simulink model "AvonGasTurbineFAult"  (R2016b)
settings: Solver=ode45  StartTime=0.0  StopTime=3000  FixedStep=1  RelTol=1e-3  EnableMultiTasking=on
InitFcn:
  | warning off
undefined symbols (not defined in the file or in its folder): flagFalut, thresholdbound, xflt
libraries: neural x74, fuzblock x6, simulink x5
(part 1 of 4)
settings Model: Creator=Me  LastModifiedBy=Ali
settings DataIOCC: LimitDataPoints=on  SaveFormat=Array  SignalLoggingSaveFormat=ModelDataLogs
settings OptimizationCC: ExpressionDepthLimit=2147483647  LifeSpan=inf
settings DebuggingCC: UnderspecifiedInitializationDetection=Classic  MergeDetectMultiDrivingBlocksExec=none  SolverPrmCheckMsg=warning  FcnCallInpInsideContextMsg=warning  StateNameClashWarn=warning  SFUnexpectedBacktrackingDiag=warning  SFNoUnconditionalDefaultTransitionDiag=warning  SFExecutionAtInitializationDiag=none
settings HardwareCC: ProdBitPerPointer=32  ProdBitPerSizeT=32  ProdBitPerPtrDiffT=32  ProdLargestAtomicFloat=None  ProdIntDivRoundTo=Undefined  ProdEndianess=Unspecified  ProdWordSize=32  ProdHWDeviceType=32-bit Generic
settings ModelReferenceCC: PropagateSignalLabelsOutOfModel=off
settings GRTTargetCC: TargetLangStandard=C89/C90 (ANSI)  GeneratePreprocessorConditionals=Disable all  CombineOutputUpdateFcns=off  GRTInterface=on
settings ConfigComp: CovMetricSettings=dw  CovHtmlReporting=on  CovSaveCumulativeToWorkspaceVar=on  CovSaveSingleToWorkspaceVar=on  CovExternalEMLEnable=off  CovSFcnEnable=off
settings ConfigurationSet: Description=SimMechanics 2G

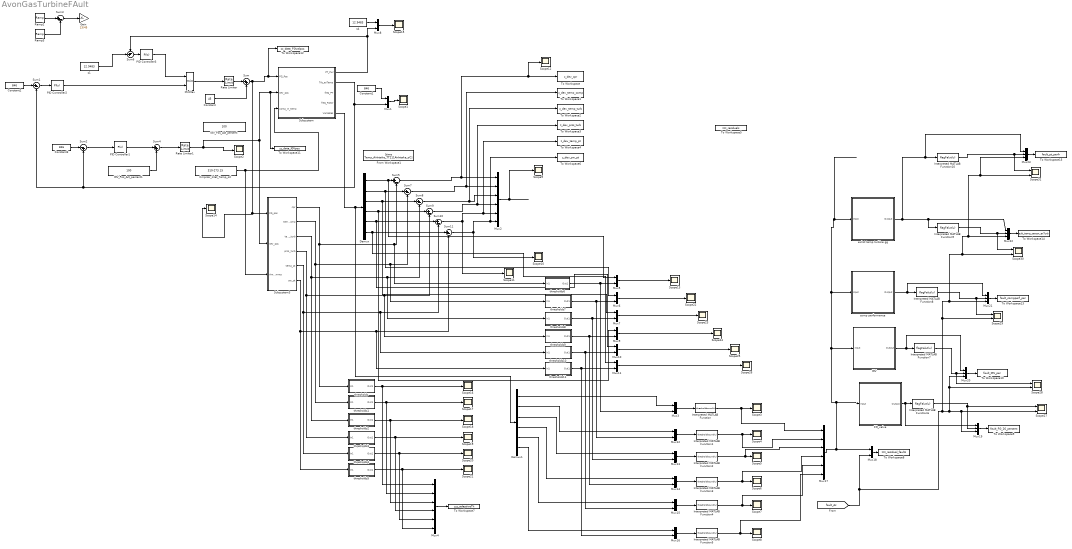
== system AvonGasTurbineFAult ==
  Cmprssr_Inlet_Temp_oC : Constant  Value=310-273.15
  Constant : Constant  Value=45
  Constant1 : Constant  Value=846
  Constant2 : Constant  Value=846
  Constant3 : Constant  Value=846
  Demux : Demux  Outputs=6
  Demux1 : Demux  Outputs=6
  FG_valve : Subsystem
      mask help: Pattern Recognition Neural Network
      mask Display: e = 0.06;c1 = [120 150 230]/255;c2 = ([120 150 230]+0)/383;c3 = ([120 150 230]+128)/383;patch([0 1 1 0],[0 0 1 1],c1);patch([0 1 1 1-e 1-e 0+e],[0 0 1 1-e 0+e 0+e],c2);patch([0 0 1 1-e 0+e 0+e],[0 1 1 1-e 1-e 0+e],c3);plot([0 1 1 0 0],[0 0 1 1 0]);fprintf('NNET');port_label('input',1,' Input');port_label('output',1,'Output ');
  From Workspace1 : FromWorkspace  VariableName="[time  Temp_AirIntake_TT211AirIntake_oC]"  SampleTime=0
  Gain : Gain  Gain=13/45
  IGV : Subsystem
      mask help: Pattern Recognition Neural Network
      mask Display: e = 0.06;c1 = [120 150 230]/255;c2 = ([120 150 230]+0)/383;c3 = ([120 150 230]+128)/383;patch([0 1 1 0],[0 0 1 1],c1);patch([0 1 1 1-e 1-e 0+e],[0 0 1 1-e 0+e 0+e],c2);patch([0 0 1 1-e 0+e 0+e],[0 1 1 1-e 1-e 0+e],c3);plot([0 1 1 0 0],[0 0 1 1 0]);fprintf('NNET');port_label('input',1,' Input');port_label('output',1,'Output ');
  IGV_Pos_Act_percent : Constant  Value=100
  IGV_Pos_Act_percent1 : Constant  Value=100
  Interpreted MATLAB Function{,1..5} (6 alike) : MATLABFcn  MATLABFcn=thresholdbound(u)  OutputDimensions=1
  Interpreted MATLAB Function{6..10} (5 alike) : MATLABFcn  MATLABFcn=flagFalut(u)  OutputDimensions=5
  MinMax : MinMax  Inputs=2
  Mux{1,3,5..16,18} (15 alike) : Mux  Inputs=2
  Mux17 : Mux  Inputs=6
  Mux{19..23} (5 alike) : Mux  Inputs=3
  Mux2 : Mux  Inputs=6
  Mux4 : Mux  Inputs=6
  PID Controller1 : simulink/Continuous/PID Controller  Controller=P  TimeDomain=Continuous-time  SampleTime=-1  IntegratorMethod=Forward Euler  FilterMethod=Forward Euler  Form=Ideal  UseFilter=on  ControllerParametersSource=internal  P=0.1  I=0.180070827922895  D=0  N=100  InitialConditionSource=internal  InitialConditionForIntegrator=0  InitialConditionForFilter=0  ExternalReset=none  LimitOutput=on  UpperSaturationLimit=15  LowerSaturationLimit=-100  LinearizeAsGain=on  AntiWindupMode=back-calculation  Kb=0.2  TrackingMode=off  Kt=1  PParamMin=[]  PParamMax=[]  IParamMin=[]  IParamMax=[]  DParamMin=[]  DParamMax=[]  NParamMin=[]  NParamMax=[]  KbParamMin=[]  KbParamMax=[]  KtParamMin=[]  KtParamMax=[]  POutMin=[]  POutMax=[]  IOutMin=[]  IOutMax=[]  DOutMin=[]  DOutMax=[]  NOutMin=[]  NOutMax=[]  KbOutMin=[]  KbOutMax=[]  KtOutMin=[]  KtOutMax=[]  IntegratorOutMin=[]  IntegratorOutMax=[]  FilterOutMin=[]  FilterOutMax=[]  SumOutMin=[]  SumOutMax=[]  SumI1OutMin=[]  SumI1OutMax=[]  SumI2OutMin=[]  SumI2OutMax=[]  SumI3OutMin=[]  SumI3OutMax=[]  SumDOutMin=[]  SumDOutMax=[]  SaturationOutMin=[]  SaturationOutMax=[]  IntegratorContinuousStateAttributes=''  IntegratorStateMustResolveToSignalObject=off  IntegratorRTWStateStorageClass=Auto  FilterContinuousStateAttributes=''  FilterStateMustResolveToSignalObject=off  FilterRTWStateStorageClass=Auto  DifferentiatorICPrevScaledInput=0  DifferentiatorOutMin=[]  DifferentiatorOutMax=[]
  PID Controller2 : simulink/Continuous/PID Controller  Controller=PI  TimeDomain=Continuous-time  SampleTime=-1  IntegratorMethod=Forward Euler  FilterMethod=Forward Euler  Form=Ideal  UseFilter=on  ControllerParametersSource=internal  P=0.0377674081389  I=0.180070827922895  D=0  N=100  InitialConditionSource=internal  InitialConditionForIntegrator=0  InitialConditionForFilter=0  ExternalReset=none  LimitOutput=on  UpperSaturationLimit=45  LowerSaturationLimit=-45  LinearizeAsGain=on  AntiWindupMode=back-calculation  Kb=0.2  TrackingMode=off  Kt=1  PParamMin=[]  PParamMax=[]  IParamMin=[]  IParamMax=[]  DParamMin=[]  DParamMax=[]  NParamMin=[]  NParamMax=[]  KbParamMin=[]  KbParamMax=[]  KtParamMin=[]  KtParamMax=[]  POutMin=[]  POutMax=[]  IOutMin=[]  IOutMax=[]  DOutMin=[]  DOutMax=[]  NOutMin=[]  NOutMax=[]  KbOutMin=[]  KbOutMax=[]  KtOutMin=[]  KtOutMax=[]  IntegratorOutMin=[]  IntegratorOutMax=[]  FilterOutMin=[]  FilterOutMax=[]  SumOutMin=[]  SumOutMax=[]  SumI1OutMin=[]  SumI1OutMax=[]  SumI2OutMin=[]  SumI2OutMax=[]  SumI3OutMin=[]  SumI3OutMax=[]  SumDOutMin=[]  SumDOutMax=[]  SaturationOutMin=[]  SaturationOutMax=[]  IntegratorContinuousStateAttributes=''  IntegratorStateMustResolveToSignalObject=off  IntegratorRTWStateStorageClass=Auto  FilterContinuousStateAttributes=''  FilterStateMustResolveToSignalObject=off  FilterRTWStateStorageClass=Auto  DifferentiatorICPrevScaledInput=0  DifferentiatorOutMin=[]  DifferentiatorOutMax=[]
  PID Controller3 : simulink/Continuous/PID Controller  Controller=PI  TimeDomain=Continuous-time  SampleTime=-1  IntegratorMethod=Forward Euler  FilterMethod=Forward Euler  Form=Ideal  UseFilter=on  ControllerParametersSource=internal  P=0.05  I=0.8  D=0  N=100  InitialConditionSource=internal  InitialConditionForIntegrator=0  InitialConditionForFilter=0  ExternalReset=none  LimitOutput=on  UpperSaturationLimit=60  LowerSaturationLimit=-30  LinearizeAsGain=on  AntiWindupMode=back-calculation  Kb=0.2  TrackingMode=off  Kt=1  PParamMin=[]  PParamMax=[]  IParamMin=[]  IParamMax=[]  DParamMin=[]  DParamMax=[]  NParamMin=[]  NParamMax=[]  KbParamMin=[]  KbParamMax=[]  KtParamMin=[]  KtParamMax=[]  POutMin=[]  POutMax=[]  IOutMin=[]  IOutMax=[]  DOutMin=[]  DOutMax=[]  NOutMin=[]  NOutMax=[]  KbOutMin=[]  KbOutMax=[]  KtOutMin=[]  KtOutMax=[]  IntegratorOutMin=[]  IntegratorOutMax=[]  FilterOutMin=[]  FilterOutMax=[]  SumOutMin=[]  SumOutMax=[]  SumI1OutMin=[]  SumI1OutMax=[]  SumI2OutMin=[]  SumI2OutMax=[]  SumI3OutMin=[]  SumI3OutMax=[]  SumDOutMin=[]  SumDOutMax=[]  SaturationOutMin=[]  SaturationOutMax=[]  IntegratorContinuousStateAttributes=''  IntegratorStateMustResolveToSignalObject=off  IntegratorRTWStateStorageClass=Auto  FilterContinuousStateAttributes=''  FilterStateMustResolveToSignalObject=off  FilterRTWStateStorageClass=Auto  DifferentiatorICPrevScaledInput=0  DifferentiatorOutMin=[]  DifferentiatorOutMax=[]
  Ramp2 : simulink/Sources/Ramp  slope=0.05  start=1000  X0=30
  Ramp3 : simulink/Sources/Ramp  slope=0.05  start=1300  X0=0
  Rate Limiter : RateLimiter  RisingSlewLimit=0.1  FallingSlewLimit=-0.1  SampleTimeMode=inherited  InitialCondition=45
  Rate Limiter1 : RateLimiter  RisingSlewLimit=0.1  FallingSlewLimit=-0.1  SampleTimeMode=inherited  InitialCondition=45
  Scope{1..26} (26 alike) : Scope
  Scope{27..31} (5 alike) : Scope  NumInputPorts=2
  Subsystem : Subsystem
  Subsystem3 : Subsystem
  Sum : Sum  Inputs=|++
  Sum{1,3,5,7..11} (8 alike) : Sum  Inputs=|+-
  Sum2 : Sum  Inputs=|-+
  Sum4 : Sum  Inputs=|++
  Sum6 : Sum  Inputs=-+|
  To Workspace : ToWorkspace  VariableName=z_dev_cpr  SampleTime=1
  To Workspace1 : ToWorkspace  VariableName=z_dev_temo_comp  SampleTime=1
  To Workspace10 : ToWorkspace  VariableName=fault_IGV_per  SampleTime=1
  To Workspace11 : ToWorkspace  VariableName=zz_data_IGVpos  SampleTime=1
  To Workspace12 : ToWorkspace  VariableName=zz_data_FGvalpos  SampleTime=1
  To Workspace13 : ToWorkspace  VariableName=fault_compperf_per  SampleTime=1
  To Workspace14 : ToWorkspace  VariableName=fault_temp_sensor_exTurb  SampleTime=1
  To Workspace15 : ToWorkspace  VariableName=fault_pt_perfr  SampleTime=1
  To Workspace2 : ToWorkspace  VariableName=z_dev_temp_turb  SampleTime=1
  To Workspace3 : ToWorkspace  VariableName=z_dev_prss_turb  SampleTime=1
  To Workspace4 : ToWorkspace  VariableName=z_dev_temp_pt  SampleTime=1
  To Workspace5 : ToWorkspace  VariableName=zzz_residuals  SampleTime=1
  To Workspace6 : ToWorkspace  VariableName=z_dev_pw_pt  SampleTime=1
  To Workspace7 : ToWorkspace  VariableName=zzz_adaptiveTh  SampleTime=1
  To Workspace8 : ToWorkspace  VariableName=zzz_residual_faults  SampleTime=1
  To Workspace9 : ToWorkspace  VariableName=fault_FG_26_percent  SampleTime=1
  comp performance : Subsystem
      mask help: Pattern Recognition Neural Network
      mask Display: e = 0.06;c1 = [120 150 230]/255;c2 = ([120 150 230]+0)/383;c3 = ([120 150 230]+128)/383;patch([0 1 1 0],[0 0 1 1],c1);patch([0 1 1 1-e 1-e 0+e],[0 0 1 1-e 0+e 0+e],c2);patch([0 0 1 1-e 0+e 0+e],[0 1 1 1-e 1-e 0+e],c3);plot([0 1 1 0 0],[0 0 1 1 0]);fprintf('NNET');port_label('input',1,' Input');port_label('output',1,'Output ');
  exhst temp turbine gg : Subsystem
      mask help: Pattern Recognition Neural Network
      mask Display: e = 0.06;c1 = [120 150 230]/255;c2 = ([120 150 230]+0)/383;c3 = ([120 150 230]+128)/383;patch([0 1 1 0],[0 0 1 1],c1);patch([0 1 1 1-e 1-e 0+e],[0 0 1 1-e 0+e 0+e],c2);patch([0 0 1 1-e 0+e 0+e],[0 1 1 1-e 1-e 0+e],c3);plot([0 1 1 0 0],[0 0 1 1 0]);fprintf('NNET');port_label('input',1,' Input');port_label('output',1,'Output ');
  s1 : Constant  Value=12.9483
  s4 : Constant  Value=12.9483
  thresholds : Subsystem
  thresholds1 : Subsystem
  thresholds10 : Subsystem
  thresholds11 : Subsystem
  thresholds2 : Subsystem
  thresholds3 : Subsystem
  thresholds4 : Subsystem
  thresholds5 : Subsystem
  thresholds6 : Subsystem
  thresholds7 : Subsystem
  thresholds8 : Subsystem
  thresholds9 : Subsystem
  wires:
  Ramp3/1 -> Sum3/2
  Ramp2/1 -> Sum3/1
  Subsystem/2(Trb_exTemp) -> Mux1/2, Sum2/2, Sum1/2
  Sum3/1 -> Gain/1
  Sum6/1 -> PID Controller3/1
  Sum1/1 -> PID Controller2/1
  Constant2/1 -> Sum1/1
  PID Controller2/1 -> MinMax/2
  MinMax/1 -> Rate Limiter/1
  PID Controller3/1 -> MinMax/1
  Mux8/1 -> Scope15/1
  s4/1 -> Mux8/1
  Subsystem/1(PT_Pwr) -> Sum6/1, Mux8/2
  Constant/1 -> Sum/2
  Sum/1 -> To Workspace12/1, Subsystem/1(FG_Pos), Scope14/1, Subsystem3/1(FG_pos)
  Rate Limiter/1 -> Sum/1
  Mux1/1 -> Scope1/1
  Constant1/1 -> Mux1/1
  Sum2/1 -> PID Controller1/1
  Constant3/1 -> Sum2/1
  PID Controller1/1 -> Sum4/1
  IGV_Pos_Act_percent1/1 -> Sum4/2
  Sum4/1 -> Rate Limiter1/1
  Rate Limiter1/1 -> Subsystem3/2(IGV_pos), To Workspace11/1, Subsystem/2(IGV_pos), Scope2/1
  Cmprssr_Inlet_Temp_oC/1 -> Subsystem3/3(Amb_Temmp), Subsystem/3(comp_in_temp)
  Subsystem3/2(temp_comp) -> thresholds7/1(In1), Sum7/2, thresholds1/1(In1)
  Subsystem3/5(temp_pt) -> thresholds10/1(In1), Sum10/2, thresholds4/1(In1)
  Subsystem3/6(pw_pt) -> thresholds11/1(In1), Sum11/2, thresholds5/1(In1)
  Subsystem/5(Variables) -> Demux1/1, Demux/1
  Demux/1 -> Mux5/1, Sum5/1
  Demux/4 -> Mux9/1, Sum9/1
  Demux/3 -> Mux7/1, Sum8/1
  Demux/2 -> Mux6/1, Sum7/1
  Demux/6 -> Mux11/1, Sum11/1
  Subsystem3/3(temp_turb) -> thresholds8/1(In1), Sum8/2, thresholds2/1(In1)
  Sum5/1 -> Mux2/1, Scope12/1, To Workspace/1
  Sum7/1 -> Mux2/2, To Workspace1/1
  Sum8/1 -> To Workspace2/1, Mux2/3
  Sum9/1 -> To Workspace3/1, Mux2/4
  Sum11/1 -> Scope10/1, To Workspace6/1, Mux2/6
  Mux2/1 -> Scope9/1
  Sum10/1 -> Scope11/1, To Workspace4/1, Mux2/5
  Subsystem3/1(cpr) -> Sum5/2, thresholds6/1(In1), thresholds/1(In1)
  s1/1 -> Sum6/2
  thresholds/1(Out1) -> Mux4/1, Scope16/1
  thresholds4/1(Out1) -> Mux4/5, Scope20/1
  thresholds3/1(Out1) -> Mux4/4, Scope19/1
  thresholds2/1(Out1) -> Mux4/3, Scope18/1
  thresholds1/1(Out1) -> Mux4/2, Scope17/1
  Mux4/1 -> To Workspace7/1
  Demux1/1 -> Mux3/1
  thresholds5/1(Out1) -> Mux4/6, Scope21/1
  Subsystem3/4(prss_turb) -> thresholds9/1(In1), Sum9/2, thresholds3/1(In1)
  thresholds6/1(Out1) -> Mux3/2, Mux5/2
  thresholds11/1(Out1) -> Mux16/2, Mux11/2
  thresholds10/1(Out1) -> Mux15/2, Mux10/2
  thresholds9/1(Out1) -> Mux14/2, Mux9/2
  thresholds8/1(Out1) -> Mux13/2, Mux7/2
  thresholds7/1(Out1) -> Mux12/2, Mux6/2
  Demux/5 -> Mux10/1, Sum10/1
  Mux5/1 -> Scope13/1
  Mux6/1 -> Scope22/1
  Mux7/1 -> Scope23/1
  Mux9/1 -> Scope24/1
  Mux10/1 -> Scope25/1
  Mux11/1 -> Scope26/1
  Demux1/2 -> Mux12/1
  Demux1/3 -> Mux13/1
  Demux1/4 -> Mux14/1
  Demux1/5 -> Mux15/1
  Demux1/6 -> Mux16/1
  Interpreted MATLAB Function1/1 -> Mux17/2, Scope4/1
  Interpreted MATLAB Function2/1 -> Mux17/3, Scope5/1
  Interpreted MATLAB Function3/1 -> Mux17/4, Scope6/1
  Interpreted MATLAB Function4/1 -> Mux17/5, Scope7/1
  Interpreted MATLAB Function5/1 -> Mux17/6, Scope8/1
  Interpreted MATLAB Function/1 -> Mux17/1, Scope3/1
  Mux3/1 -> Interpreted MATLAB Function/1
  Mux12/1 -> Interpreted MATLAB Function1/1
  Mux13/1 -> Interpreted MATLAB Function2/1
  Mux14/1 -> Interpreted MATLAB Function3/1
  Mux15/1 -> Interpreted MATLAB Function4/1
  Mux16/1 -> Interpreted MATLAB Function5/1
  Mux18/1 -> To Workspace8/1
  FG_valve/1(Output) -> Mux19/1, Interpreted MATLAB Function6/1
  Mux17/1 -> Mux18/1, FG_valve/1(Input), IGV/1(Input), exhst temp turbine gg/1(Input), comp performance/1(Input)
  Interpreted MATLAB Function6/1 -> Mux19/2, Scope27/1
  Mux19/1 -> To Workspace9/1
  IGV/1(Output) -> Mux20/1, Interpreted MATLAB Function7/1
  Mux20/1 -> To Workspace10/1
  Interpreted MATLAB Function7/1 -> Scope28/1, Mux20/2
  comp performance/1(Output) -> Mux21/1, Interpreted MATLAB Function8/1
  Mux21/1 -> To Workspace13/1
  Interpreted MATLAB Function8/1 -> Scope29/1, Mux21/2
  Mux22/1 -> To Workspace14/1
  Interpreted MATLAB Function9/1 -> Mux22/2, Scope30/1
  exhst temp turbine gg/1(Output) -> Interpreted MATLAB Function10/1, Mux23/1, Interpreted MATLAB Function9/1, Mux22/1
  Mux23/1 -> To Workspace15/1
  [fault_Ac] -> Scope29/2, Scope31/2, Mux23/3, Mux22/3, Scope30/2, Mux21/3, Scope28/2, Mux20/3, Mux19/3, Scope27/2, Mux18/2
  Interpreted MATLAB Function10/1 -> Scope31/1, Mux23/2

== system AvonGasTurbineFAult/FG_valve ==
  Input : Inport  PortDimensions=6
      mask Display: e = 0.06;c1 = [120 230 180]/255;c2 = ([120 230 180]+0)/(256+128);c3 = ([120 230 180]+128)/(256+128);patch([0 1 1 0],[0 0 1 1],c1);patch([0 1 1 1-e 1-e 0+e],[0 0 1 1-e 0+e 0+e],c2);patch([0 0 1 1-e 0+e 0+e],[0 1 1 1-e 1-e 0+e],c3);plot([0 1 1 0 0],[0 0 1 1 0]);
  Layer 1 : Subsystem
      mask Display: e = 0.06;c1 = [120 150 230]/255;c2 = ([120 150 230]+0)/383;c3 = ([120 150 230]+128)/383;patch([0 1 1 0],[0 0 1 1],c1);patch([0 1 1 1-e 1-e 0+e],[0 0 1 1-e 0+e 0+e],c2);patch([0 0 1 1-e 0+e 0+e],[0 1 1 1-e 1-e 0+e],c3);plot([0 1 1 0 0],[0 0 1 1 0]);
  Layer 2 : Subsystem
      mask Display: e = 0.06;c1 = [120 150 230]/255;c2 = ([120 150 230]+0)/383;c3 = ([120 150 230]+128)/383;patch([0 1 1 0],[0 0 1 1],c1);patch([0 1 1 1-e 1-e 0+e],[0 0 1 1-e 0+e 0+e],c2);patch([0 0 1 1-e 0+e 0+e],[0 1 1 1-e 1-e 0+e],c3);plot([0 1 1 0 0],[0 0 1 1 0]);
  Process Input 1 : Subsystem
      mask Display: e = 0.06;c1 = [120 150 230]/255;c2 = ([120 150 230]+0)/383;c3 = ([120 150 230]+128)/383;patch([0 1 1 0],[0 0 1 1],c1);patch([0 1 1 1-e 1-e 0+e],[0 0 1 1-e 0+e 0+e],c2);patch([0 0 1 1-e 0+e 0+e],[0 1 1 1-e 1-e 0+e],c3);plot([0 1 1 0 0],[0 0 1 1 0]);
  Process Output 1 : Subsystem
      mask Display: e = 0.06;c1 = [120 150 230]/255;c2 = ([120 150 230]+0)/383;c3 = ([120 150 230]+128)/383;patch([0 1 1 0],[0 0 1 1],c1);patch([0 1 1 1-e 1-e 0+e],[0 0 1 1-e 0+e 0+e],c2);patch([0 0 1 1-e 0+e 0+e],[0 1 1 1-e 1-e 0+e],c3);plot([0 1 1 0 0],[0 0 1 1 0]);
  Output : Outport  InitialOutput=[0;0;0;0;0]
      mask Display: e = 0.06;c1 = [120 230 180]/255;c2 = ([120 230 180]+0)/(256+128);c3 = ([120 230 180]+128)/(256+128);patch([0 1 1 0],[0 0 1 1],c1);patch([0 1 1 1-e 1-e 0+e],[0 0 1 1-e 0+e 0+e],c2);patch([0 0 1 1-e 0+e 0+e],[0 1 1 1-e 1-e 0+e],c3);plot([0 1 1 0 0],[0 0 1 1 0]);
  wires:
  Input/1 -> Process Input 1/1(x)
  Process Output 1/1(y) -> Output/1
  Process Input 1/1(p) -> Layer 1/1("p{1}")
  Layer 1/1("a{1}") -> [feedback1]
  [feedback1] -> Layer 2/1("a{1} ")
  Layer 2/1("a{2}") -> Process Output 1/1(a)

== system AvonGasTurbineFAult/IGV ==
  Input : Inport  PortDimensions=6
      mask Display: e = 0.06;c1 = [120 230 180]/255;c2 = ([120 230 180]+0)/(256+128);c3 = ([120 230 180]+128)/(256+128);patch([0 1 1 0],[0 0 1 1],c1);patch([0 1 1 1-e 1-e 0+e],[0 0 1 1-e 0+e 0+e],c2);patch([0 0 1 1-e 0+e 0+e],[0 1 1 1-e 1-e 0+e],c3);plot([0 1 1 0 0],[0 0 1 1 0]);
  Layer 1 : Subsystem
      mask Display: e = 0.06;c1 = [120 150 230]/255;c2 = ([120 150 230]+0)/383;c3 = ([120 150 230]+128)/383;patch([0 1 1 0],[0 0 1 1],c1);patch([0 1 1 1-e 1-e 0+e],[0 0 1 1-e 0+e 0+e],c2);patch([0 0 1 1-e 0+e 0+e],[0 1 1 1-e 1-e 0+e],c3);plot([0 1 1 0 0],[0 0 1 1 0]);
  Layer 2 : Subsystem
      mask Display: e = 0.06;c1 = [120 150 230]/255;c2 = ([120 150 230]+0)/383;c3 = ([120 150 230]+128)/383;patch([0 1 1 0],[0 0 1 1],c1);patch([0 1 1 1-e 1-e 0+e],[0 0 1 1-e 0+e 0+e],c2);patch([0 0 1 1-e 0+e 0+e],[0 1 1 1-e 1-e 0+e],c3);plot([0 1 1 0 0],[0 0 1 1 0]);
  Process Input 1 : Subsystem
      mask Display: e = 0.06;c1 = [120 150 230]/255;c2 = ([120 150 230]+0)/383;c3 = ([120 150 230]+128)/383;patch([0 1 1 0],[0 0 1 1],c1);patch([0 1 1 1-e 1-e 0+e],[0 0 1 1-e 0+e 0+e],c2);patch([0 0 1 1-e 0+e 0+e],[0 1 1 1-e 1-e 0+e],c3);plot([0 1 1 0 0],[0 0 1 1 0]);
  Process Output 1 : Subsystem
      mask Display: e = 0.06;c1 = [120 150 230]/255;c2 = ([120 150 230]+0)/383;c3 = ([120 150 230]+128)/383;patch([0 1 1 0],[0 0 1 1],c1);patch([0 1 1 1-e 1-e 0+e],[0 0 1 1-e 0+e 0+e],c2);patch([0 0 1 1-e 0+e 0+e],[0 1 1 1-e 1-e 0+e],c3);plot([0 1 1 0 0],[0 0 1 1 0]);
  Output : Outport  InitialOutput=[0;0;0;0;0]
      mask Display: e = 0.06;c1 = [120 230 180]/255;c2 = ([120 230 180]+0)/(256+128);c3 = ([120 230 180]+128)/(256+128);patch([0 1 1 0],[0 0 1 1],c1);patch([0 1 1 1-e 1-e 0+e],[0 0 1 1-e 0+e 0+e],c2);patch([0 0 1 1-e 0+e 0+e],[0 1 1 1-e 1-e 0+e],c3);plot([0 1 1 0 0],[0 0 1 1 0]);
  wires:
  Input/1 -> Process Input 1/1(x)
  Process Output 1/1(y) -> Output/1
  Process Input 1/1(p) -> Layer 1/1("p{1}")
  Layer 1/1("a{1}") -> [feedback1]
  [feedback1] -> Layer 2/1("a{1} ")
  Layer 2/1("a{2}") -> Process Output 1/1(a)

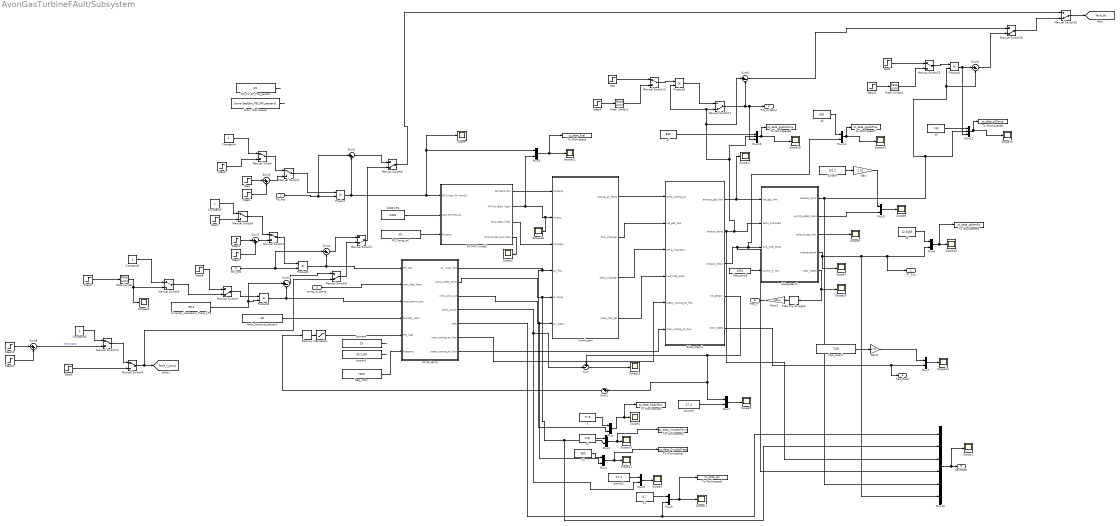
== system AvonGasTurbineFAult/Subsystem ==
  FG_Pos : Inport
  IGV_pos : Inport  Port=2
  comp_in_temp : Inport  Port=3
  2400 kPa : Constant  Value=2400
  Amb_Moisture_percent : Constant  Value=65
  Cmprssr_Upstream_Press_kPa : Constant  Value=99.2
  Combustor : Subsystem
  Constant{2..5} (4 alike) : Constant
  ExhaPr : Constant  Value=101.2
  FG MCV model : Subsystem
  FG_CV_SP_Pos_percen : Constant  Value=45
  FG_Temp_oC : Constant  Value=20
  From Workspace : FromWorkspace  VariableName=[time GasGen_PID_MV_percent]  SampleTime=0
  Gain : Gain  Gain=2.01
  Gain1 : Gain  Gain=30/pi
  Gain2 : Gain  Gain=pi/30
  Manual Switch{,1..2,4..5,9,12..13,15} (9 alike) : ManualSwitch
  Manual Switch{3,6..8,10..11,16} (7 alike) : ManualSwitch  CurrentSetting=0
  Memory : Memory  X0=28.945
  Memory Omega2 : Memory  X0=pi/30*4901
  Mux{,1..9,11} (11 alike) : Mux  Inputs=2
  Mux10 : Mux  Inputs=3
  Mux12 : Mux  Inputs=3
  Mux13 : Mux  Inputs=6
  Product{,1..4} (5 alike) : Product
  Rate Limiter : RateLimiter  RisingSlewLimit=0.005  FallingSlewLimit=-0.005  SampleTimeMode=inherited
  Rate Limiter1 : RateLimiter  RisingSlewLimit=0.005  FallingSlewLimit=-0.005  SampleTimeMode=inherited
  Rate Limiter2 : RateLimiter  RisingSlewLimit=0.005  FallingSlewLimit=-0.005  SampleTimeMode=inherited
  Saturation : Saturate  UpperLimit=40  LowerLimit=1
  Scope{,1..4,6..23} (23 alike) : Scope
  Step{,2..3,5,9,11} (6 alike) : Step  Time=1500  Before=1  After=1-xflt  SampleTime=0
  Step1 : Step  Time=1700  After=xflt  SampleTime=0
  Step10 : Step  Time=1200  Before=1  After=0.97  SampleTime=0
  Step12 : Step  Time=2000  After=-0.02  SampleTime=0
  Step4 : Step  Time=1700  After=xflt  SampleTime=0
  Step6 : Step  Time=1500  Before=1  After=0.976  SampleTime=0
  Step7 : Step  Time=1200  Before=1  After=1-0.09  SampleTime=0
  Step8 : Step  Time=1200  Before=1  After=1-0.07  SampleTime=0
  Subsystem1 : Subsystem
  Subsystem2 : Subsystem
  Sum : Sum  Inputs=+-|
  Sum1 : Sum  Inputs=-+|
  Sum{2,4..6,9} (5 alike) : Sum  Inputs=|+-
  Sum3 : Sum  Inputs=|++
  Sum7 : Sum  Inputs=|++
  Sum8 : Sum  Inputs=|++
  To Workspace : ToWorkspace  VariableName=zz_data_fuel  SampleTime=1
  To Workspace1 : ToWorkspace  VariableName=zz_data_cpr  SampleTime=1
  To Workspace2 : ToWorkspace  VariableName=zz_data_CmpdisPress  SampleTime=1
  To Workspace3 : ToWorkspace  VariableName=zz_data_CmpdisTemp  SampleTime=1
  To Workspace4 : ToWorkspace  VariableName=zz_data_trbAirflow  SampleTime=1
  To Workspace5 : ToWorkspace  VariableName=zz_data_ptGenPw  SampleTime=1
  To Workspace6 : ToWorkspace  VariableName=zz_data_ggdisTemp  SampleTime=1
  To Workspace7 : ToWorkspace  VariableName=zz_data_ggdisPres  SampleTime=1
  To Workspace8 : ToWorkspace  VariableName=zz_data_ptTemp  SampleTime=1
  comp_temp : Subsystem
  freq_pwtrb : Constant  Value=4901
  freq_rotor : Constant  Value=7250
  freq_rotor1 : Constant  Value=7250
  power2 : Constant  Value=27.4
  power4 : Constant  Value=25
  power5 : Constant  Value=26.2350
  power6 : Constant  Value=27.4
  s : Constant  Value=77.8
  s1 : Constant  Value=9.7
  s2 : Constant  Value=378
  s3 : Constant  Value=960
  s4 : Constant  Value=12.9483
  s7 : Constant  Value=846
  s8 : Constant  Value=335
  s9 : Constant  Value=745
  test : Step  Time=1200  Before=1  After=0.95  SampleTime=0
  test1 : Step  Time=1200  Before=1  After=0.95  SampleTime=0
  PT_Pwr : Outport
  Trb_exTemp : Outport  Port=2
  freq_PT : Outport  Port=3
  freq_Rotor : Outport  Port=4
  Variables : Outport  Port=5
  tag scope: fault_Ac=global, fault_f_comp=global
  wires:
  FG_CV_SP_Pos_percen/1 -> ?
  From Workspace/1 -> ?
  Gain1/1 -> freq_PT/1
  power5/1 -> ?
  power4/1 -> ?
  Amb_Moisture_percent/1 -> comp_temp/4(humidity_ratio)
  freq_rotor/1 -> comp_temp/6(Frequency)
  IGV_pos/1 -> Product1/2, Sum4/1
  Subsystem1/3(exhaust_gas_flow) -> Scope6/1
  Memory/1 -> Saturation/1
  FG_Temp_oC/1 -> FG MCV model/3(FG temp.)
  comp_temp/3(comp_prss_out) -> Mux4/2, Combustor/6(air_press)
  FG MCV model/2(FG Flow @bur (kg/s)) -> Mux9/2, Scope16/1, Combustor/2(FG flow)
  Combustor/2(flow_chamber) -> Subsystem2/2(hot_gas_flow)
  comp_temp/4(comp_power) -> Mux5/2, Sum/2
  Mux1/1 -> Scope9/1
  Mux6/1 -> To Workspace1/1, Scope11/1
  comp_temp/5(CPR) -> Mux13/1, Mux6/2
  Mux4/1 -> To Workspace2/1, Scope12/1
  FG MCV model/1(FG Temp (oC)) -> Combustor/1(FG temp)
  Mux2/1 -> To Workspace3/1, Scope10/1
  2400 kPa/1 -> FG MCV model/2(main FG line prss)
  ExhaPr/1 -> Gain/1
  Combustor/1(cooling_air_temp) -> Subsystem2/1(temp_cooling_air)
  FG MCV model/3(FG pr @bur (kPa)) -> Combustor/3(FG press)
  Subsystem2/3(exhaust_press) -> Mux13/4, Subsystem1/3(turb_inlet_press), Mux11/2
  Combustor/3(temp_chamber) -> Subsystem2/3(temp_chambers)
  FG MCV model/4(FG skid inlet prss (kPa)) -> Scope2/1
  Subsystem2/1(exhaust_gas_flow) -> Subsystem1/1(hot_gas_flow), Scope17/1
  Subsystem1/2(pwrtrb_outlet_press) -> Mux3/2
  power6/1 -> Mux1/2
  Gain/1 -> Mux3/1
  Mux3/1 -> Scope8/1
  comp_temp/1(air_mass_flow) -> Combustor/4(air_flow), Mux/2
  comp_temp/2(comp_outlet_temp) -> Mux13/2, Mux2/2, Combustor/5(air temp)
  Combustor/4(press_hot_gas) -> Subsystem2/4(turb_inlet_press)
  Mux8/1 -> To Workspace5/1, Scope15/1
  Mux7/1 -> Scope14/1
  Product/1 -> Mux9/1, Scope/1, FG MCV model/1(FG CV pos (%) chmb1), Sum2/2
  Subsystem1/4(turbine_power) -> Mux13/6, PT_Pwr/1, Mux8/2, Scope7/1
  comp_temp/7(stator_cooling_air_flow) -> Subsystem2/6(rotor_cooling_air_flow)
  Mux11/1 -> To Workspace7/1, Scope22/1
  s2/1 -> Mux2/1
  Sum1/1 -> Memory/1
  Mux9/1 -> To Workspace/1, Scope21/1
  Mux/1 -> To Workspace4/1, Scope4/1
  s/1 -> Mux/1
  s7/1 -> Mux10/1
  s1/1 -> Mux6/1
  Mux10/1 -> Scope18/1, To Workspace6/1
  Mux5/1 -> Scope3/1
  Sum/1 -> Scope13/1
  Subsystem2/5(rotor_speed) -> freq_Rotor/1, Mux7/2
  comp_temp/6(rotor_cooling_air_flow) -> Subsystem2/5(stator_cooling_air_flow)
  s3/1 -> Mux4/1
  freq_pwtrb/1 -> Subsystem1/4(pwrtrb_fr_rpm)
  power2/1 -> Mux5/1
  Subsystem1/5(rotor_speed) -> Scope20/1, Memory Omega2/1
  Gain2/1 -> Mux7/1
  Saturation/1 -> comp_temp/5(MW_load)
  Memory Omega2/1 -> Gain1/1
  freq_rotor1/1 -> Gain2/1
  Subsystem2/4(trb_genpwr) -> Sum/1, Sum1/2, Mux1/1
  s4/1 -> Mux8/1
  s9/1 -> Mux12/1
  s8/1 -> Mux11/1
  Mux12/1 -> To Workspace8/1, Scope19/1
  comp_in_temp/1 -> comp_temp/2(cmp_Inlet_Temp)
  FG_Pos/1 -> Sum2/1, Product/2
  Mux13/1 -> Scope1/1, Variables/1
  Sum2/1 -> Manual Switch6/1
  Step/1 -> Sum3/1
  Step1/1 -> Sum3/2
  Product1/1 -> Sum4/2, comp_temp/1(IGV_pos)
  Manual Switch5/1 -> Manual Switch2/1
  Cmprssr_Upstream_Press_kPa/1 -> Sum5/1, Product2/2
  Product2/1 -> Sum5/2, comp_temp/3(cmp_upstrm_prss)
  Step2/1 -> Rate Limiter/1
  Rate Limiter/1 -> Manual Switch9/2, Scope23/1
  Step3/1 -> Sum7/1
  Step4/1 -> Sum7/2
  Manual Switch3/1 -> Product2/1
  Constant3/1 -> Manual Switch12/1
  Step6/1 -> Manual Switch/2
  Sum3/1 -> Manual Switch1/2
  Manual Switch/1 -> Manual Switch1/1
  Constant4/1 -> Manual Switch/1
  Manual Switch1/1 -> Product/1
  Manual Switch2/1 -> Product1/1
  Sum7/1 -> Manual Switch2/2
  Step8/1 -> Manual Switch3/1
  Manual Switch4/1 -> Manual Switch8/2, [fault_f_comp]
  Step5/1 -> Manual Switch4/2
  Step7/1 -> Manual Switch5/2
  Constant5/1 -> Manual Switch5/1
  Manual Switch7/1 -> Manual Switch6/2
  Manual Switch6/1 -> Manual Switch10/1
  Sum4/1 -> Manual Switch7/1
  Sum5/1 -> Manual Switch8/1
  Manual Switch8/1 -> Manual Switch7/2
  Manual Switch9/1 -> Manual Switch3/2
  Constant2/1 -> Manual Switch9/1
  Manual Switch10/1 -> [fault_Ac]
  Sum6/1 -> Manual Switch16/1
  Rate Limiter1/1 -> Manual Switch13/2
  Product3/1 -> Manual Switch11/1
  Subsystem2/2(exhaust_temp) -> Mux13/3, Sum6/1, Manual Switch11/2, Product3/2, Mux10/2, Subsystem1/2(temp_chambers)
  Manual Switch11/1 -> Mux10/3, Trb_exTemp/1, Sum6/2
  Manual Switch12/1 -> Manual Switch4/1
  Manual Switch13/1 -> Product3/1
  test/1 -> Manual Switch13/1
  Step10/1 -> Sum8/1
  Step12/1 -> Sum8/2
  Sum8/1 -> Manual Switch12/2  "test signal"
  Step9/1 -> Rate Limiter1/1
  Manual Switch16/1 -> Manual Switch10/2
  Rate Limiter2/1 -> Manual Switch15/2
  Product4/1 -> Mux12/3, Sum9/1
  Subsystem1/1(exhaust_temp) -> Mux12/2, Sum9/2, Product4/2, Mux13/5
  Manual Switch15/1 -> Product4/1
  test1/1 -> Manual Switch15/1
  Step11/1 -> Rate Limiter2/1
  Sum9/1 -> Manual Switch16/2

== system AvonGasTurbineFAult/Subsystem3 ==
  FG_pos : Inport
  IGV_pos : Inport  Port=2
  Amb_Temmp : Inport  Port=3
  CPR : fuzblock/Fuzzy Logic  Controller  fis=readfis('fis_CPR')
  Gain1 : Gain  Gain=11.0390
  Gain10 : Gain  Gain=1/115
  Gain11 : Gain  Gain=1/40
  Gain12 : Gain  Gain=888.3645
  Gain13 : Gain  Gain=381.1970
  Gain14 : Gain  Gain=779.6646
  Gain15 : Gain  Gain=17.9878
  Gain2 : Gain  Gain=382.2652
  Gain3 : Gain  Gain=1/6.6359
  Gain9 : Gain  Gain=1/50
  Laguerre3 : Subsystem  mask{a1=0.96, fltrordr=5, smp=1}
      mask prompts: a1 "Laguerre pole"; fltrordr "filter order (n=L+1)"; smp "sample time"
      mask Display: disp('Laguerre Filter')
  Laguerre4 : Subsystem  mask{a1=0.96, fltrordr=5, smp=1}
      mask prompts: a1 "Laguerre pole"; fltrordr "filter order (n=L+1)"; smp "sample time"
      mask Display: disp('Laguerre Filter')
  Laguerre5 : Subsystem  mask{a1=0.96, fltrordr=5, smp=1}
      mask prompts: a1 "Laguerre pole"; fltrordr "filter order (n=L+1)"; smp "sample time"
      mask Display: disp('Laguerre Filter')
  Mux22 : Mux  Inputs=3
  power_pt : fuzblock/Fuzzy Logic  Controller  fis=readfis('fis_power_pt')
  prss_turb1 : fuzblock/Fuzzy Logic  Controller  fis=readfis('fis_prss_turb')
  temp_comp1 : fuzblock/Fuzzy Logic  Controller  fis=readfis('fis_temp_comp')
  temp_pt1 : fuzblock/Fuzzy Logic  Controller  fis=readfis('fis_temp_pt')
  temp_turb1 : fuzblock/Fuzzy Logic  Controller  fis=readfis('fis_temp_turb')
  cpr : Outport
  temp_comp : Outport  Port=2
  temp_turb : Outport  Port=3
  prss_turb : Outport  Port=4
  temp_pt : Outport  Port=5
  pw_pt : Outport  Port=6
  wires:
  IGV_pos/1 -> Gain10/1
  Gain10/1 -> Laguerre4/1(u)
  Laguerre5/1(v) -> Mux22/3
  Gain9/1 -> Laguerre3/1(u)
  Laguerre3/1(v) -> Mux22/1
  Gain11/1 -> Laguerre5/1(u)
  Mux22/1 -> Gain3/1
  Laguerre4/1(v) -> Mux22/2
  FG_pos/1 -> Gain9/1
  Amb_Temmp/1 -> Gain11/1
  Gain1/1 -> cpr/1
  Gain2/1 -> temp_comp/1
  Gain12/1 -> temp_turb/1
  Gain13/1 -> prss_turb/1
  Gain14/1 -> temp_pt/1
  Gain15/1 -> pw_pt/1
  temp_comp1/1 -> Gain2/1
  temp_turb1/1 -> Gain12/1
  prss_turb1/1 -> Gain13/1
  temp_pt1/1 -> Gain14/1
  power_pt/1 -> Gain15/1
  CPR/1 -> Gain1/1
  Gain3/1 -> temp_turb1/1, prss_turb1/1, temp_pt1/1, power_pt/1, temp_comp1/1, CPR/1

== system AvonGasTurbineFAult/comp performance ==
  Input : Inport  PortDimensions=6
      mask Display: e = 0.06;c1 = [120 230 180]/255;c2 = ([120 230 180]+0)/(256+128);c3 = ([120 230 180]+128)/(256+128);patch([0 1 1 0],[0 0 1 1],c1);patch([0 1 1 1-e 1-e 0+e],[0 0 1 1-e 0+e 0+e],c2);patch([0 0 1 1-e 0+e 0+e],[0 1 1 1-e 1-e 0+e],c3);plot([0 1 1 0 0],[0 0 1 1 0]);
  Layer 1 : Subsystem
      mask Display: e = 0.06;c1 = [120 150 230]/255;c2 = ([120 150 230]+0)/383;c3 = ([120 150 230]+128)/383;patch([0 1 1 0],[0 0 1 1],c1);patch([0 1 1 1-e 1-e 0+e],[0 0 1 1-e 0+e 0+e],c2);patch([0 0 1 1-e 0+e 0+e],[0 1 1 1-e 1-e 0+e],c3);plot([0 1 1 0 0],[0 0 1 1 0]);
  Layer 2 : Subsystem
      mask Display: e = 0.06;c1 = [120 150 230]/255;c2 = ([120 150 230]+0)/383;c3 = ([120 150 230]+128)/383;patch([0 1 1 0],[0 0 1 1],c1);patch([0 1 1 1-e 1-e 0+e],[0 0 1 1-e 0+e 0+e],c2);patch([0 0 1 1-e 0+e 0+e],[0 1 1 1-e 1-e 0+e],c3);plot([0 1 1 0 0],[0 0 1 1 0]);
  Process Input 1 : Subsystem
      mask Display: e = 0.06;c1 = [120 150 230]/255;c2 = ([120 150 230]+0)/383;c3 = ([120 150 230]+128)/383;patch([0 1 1 0],[0 0 1 1],c1);patch([0 1 1 1-e 1-e 0+e],[0 0 1 1-e 0+e 0+e],c2);patch([0 0 1 1-e 0+e 0+e],[0 1 1 1-e 1-e 0+e],c3);plot([0 1 1 0 0],[0 0 1 1 0]);
  Process Output 1 : Subsystem
      mask Display: e = 0.06;c1 = [120 150 230]/255;c2 = ([120 150 230]+0)/383;c3 = ([120 150 230]+128)/383;patch([0 1 1 0],[0 0 1 1],c1);patch([0 1 1 1-e 1-e 0+e],[0 0 1 1-e 0+e 0+e],c2);patch([0 0 1 1-e 0+e 0+e],[0 1 1 1-e 1-e 0+e],c3);plot([0 1 1 0 0],[0 0 1 1 0]);
  Output : Outport  InitialOutput=[0;0;0;0;0]
      mask Display: e = 0.06;c1 = [120 230 180]/255;c2 = ([120 230 180]+0)/(256+128);c3 = ([120 230 180]+128)/(256+128);patch([0 1 1 0],[0 0 1 1],c1);patch([0 1 1 1-e 1-e 0+e],[0 0 1 1-e 0+e 0+e],c2);patch([0 0 1 1-e 0+e 0+e],[0 1 1 1-e 1-e 0+e],c3);plot([0 1 1 0 0],[0 0 1 1 0]);
  wires:
  Input/1 -> Process Input 1/1(x)
  Process Output 1/1(y) -> Output/1
  Process Input 1/1(p) -> Layer 1/1("p{1}")
  Layer 1/1("a{1}") -> [feedback1]
  [feedback1] -> Layer 2/1("a{1} ")
  Layer 2/1("a{2}") -> Process Output 1/1(a)

== system AvonGasTurbineFAult/exhst temp turbine gg ==
  Input : Inport  PortDimensions=6
      mask Display: e = 0.06;c1 = [120 230 180]/255;c2 = ([120 230 180]+0)/(256+128);c3 = ([120 230 180]+128)/(256+128);patch([0 1 1 0],[0 0 1 1],c1);patch([0 1 1 1-e 1-e 0+e],[0 0 1 1-e 0+e 0+e],c2);patch([0 0 1 1-e 0+e 0+e],[0 1 1 1-e 1-e 0+e],c3);plot([0 1 1 0 0],[0 0 1 1 0]);
  Layer 1 : Subsystem
      mask Display: e = 0.06;c1 = [120 150 230]/255;c2 = ([120 150 230]+0)/383;c3 = ([120 150 230]+128)/383;patch([0 1 1 0],[0 0 1 1],c1);patch([0 1 1 1-e 1-e 0+e],[0 0 1 1-e 0+e 0+e],c2);patch([0 0 1 1-e 0+e 0+e],[0 1 1 1-e 1-e 0+e],c3);plot([0 1 1 0 0],[0 0 1 1 0]);
  Layer 2 : Subsystem
      mask Display: e = 0.06;c1 = [120 150 230]/255;c2 = ([120 150 230]+0)/383;c3 = ([120 150 230]+128)/383;patch([0 1 1 0],[0 0 1 1],c1);patch([0 1 1 1-e 1-e 0+e],[0 0 1 1-e 0+e 0+e],c2);patch([0 0 1 1-e 0+e 0+e],[0 1 1 1-e 1-e 0+e],c3);plot([0 1 1 0 0],[0 0 1 1 0]);
  Process Input 1 : Subsystem
      mask Display: e = 0.06;c1 = [120 150 230]/255;c2 = ([120 150 230]+0)/383;c3 = ([120 150 230]+128)/383;patch([0 1 1 0],[0 0 1 1],c1);patch([0 1 1 1-e 1-e 0+e],[0 0 1 1-e 0+e 0+e],c2);patch([0 0 1 1-e 0+e 0+e],[0 1 1 1-e 1-e 0+e],c3);plot([0 1 1 0 0],[0 0 1 1 0]);
  Process Output 1 : Subsystem
      mask Display: e = 0.06;c1 = [120 150 230]/255;c2 = ([120 150 230]+0)/383;c3 = ([120 150 230]+128)/383;patch([0 1 1 0],[0 0 1 1],c1);patch([0 1 1 1-e 1-e 0+e],[0 0 1 1-e 0+e 0+e],c2);patch([0 0 1 1-e 0+e 0+e],[0 1 1 1-e 1-e 0+e],c3);plot([0 1 1 0 0],[0 0 1 1 0]);
  Output : Outport  InitialOutput=[0;0;0;0;0]
      mask Display: e = 0.06;c1 = [120 230 180]/255;c2 = ([120 230 180]+0)/(256+128);c3 = ([120 230 180]+128)/(256+128);patch([0 1 1 0],[0 0 1 1],c1);patch([0 1 1 1-e 1-e 0+e],[0 0 1 1-e 0+e 0+e],c2);patch([0 0 1 1-e 0+e 0+e],[0 1 1 1-e 1-e 0+e],c3);plot([0 1 1 0 0],[0 0 1 1 0]);
  wires:
  Input/1 -> Process Input 1/1(x)
  Process Output 1/1(y) -> Output/1
  Process Input 1/1(p) -> Layer 1/1("p{1}")
  Layer 1/1("a{1}") -> [feedback1]
  [feedback1] -> Layer 2/1("a{1} ")
  Layer 2/1("a{2}") -> Process Output 1/1(a)

== system AvonGasTurbineFAult/thresholds ==
  In1 : Inport
  Constant5 : Constant  Value=0.0178
  Mux5 : Mux  Inputs=3
  Sum12 : Sum  Inputs=|++
  Sum13 : Sum  Inputs=|++
  Sum14 : Sum  Inputs=-+|
  var : Gain  Gain=0.0665
  var1 : Gain  Gain=0.2
  Out1 : Outport
  wires:
  var1/1 -> var/1
  Sum14/1 -> Mux5/3
  Sum13/1 -> Sum12/1, var1/1, Sum14/2
  var/1 -> Sum14/1, Sum12/2
  Mux5/1 -> Out1/1
  Sum12/1 -> Mux5/2
  Constant5/1 -> Sum13/2
  In1/1 -> Mux5/1, Sum13/1

== system AvonGasTurbineFAult/thresholds1 ==
  In1 : Inport
  Constant5 : Constant  Value=-2.9
  Mux5 : Mux  Inputs=3
  Sum12 : Sum  Inputs=|++
  Sum13 : Sum  Inputs=|++
  Sum14 : Sum  Inputs=-+|
  var : Gain  Gain=0.0069
  var1 : Gain  Gain=2.5
  Out1 : Outport
  wires:
  In1/1 -> Sum13/1, Mux5/1
  Constant5/1 -> Sum13/2
  Sum12/1 -> Mux5/2
  Mux5/1 -> Out1/1
  var/1 -> Sum12/2, Sum14/1
  Sum13/1 -> Sum14/2, var1/1, Sum12/1
  Sum14/1 -> Mux5/3
  var1/1 -> var/1

== system AvonGasTurbineFAult/thresholds10 ==
  In1 : Inport
  Constant5 : Constant  Value=-2.0766
  Mux5 : Mux  Inputs=2
  Sum12 : Sum  Inputs=|++
  Sum13 : Sum  Inputs=|++
  Sum14 : Sum  Inputs=-+|
  var : Gain  Gain=0.03
  var1 : Gain  Gain=0.19
  Out1 : Outport
  wires:
  var1/1 -> var/1
  Sum14/1 -> Mux5/2
  Sum13/1 -> Sum12/1, var1/1, Sum14/2
  var/1 -> Sum14/1, Sum12/2
  Mux5/1 -> Out1/1
  Sum12/1 -> Mux5/1
  Constant5/1 -> Sum13/2
  In1/1 -> Sum13/1

== system AvonGasTurbineFAult/thresholds11 ==
  In1 : Inport
  Constant5 : Constant  Value=0
  Mux5 : Mux  Inputs=2
  Sum12 : Sum  Inputs=|++
  Sum13 : Sum  Inputs=|++
  Sum14 : Sum  Inputs=-+|
  var : Gain  Gain=0.25
  var1 : Gain  Gain=0.22
  Out1 : Outport
  wires:
  In1/1 -> Sum13/1
  Constant5/1 -> Sum13/2
  Sum12/1 -> Mux5/1
  Mux5/1 -> Out1/1
  var/1 -> Sum12/2, Sum14/1
  Sum13/1 -> Sum14/2, var1/1, Sum12/1
  Sum14/1 -> Mux5/2
  var1/1 -> var/1

== system AvonGasTurbineFAult/thresholds2 ==
  In1 : Inport
  Constant5 : Constant  Value=0.05
  Mux5 : Mux  Inputs=3
  Sum12 : Sum  Inputs=|++
  Sum13 : Sum  Inputs=|++
  Sum14 : Sum  Inputs=-+|
  var : Gain  Gain=0.05
  var1 : Gain  Gain=0.19
  Out1 : Outport
  wires:
  var1/1 -> var/1
  Sum14/1 -> Mux5/3
  Sum13/1 -> Sum12/1, var1/1, Sum14/2
  var/1 -> Sum14/1, Sum12/2
  Mux5/1 -> Out1/1
  Sum12/1 -> Mux5/2
  Constant5/1 -> Sum13/2
  In1/1 -> Mux5/1, Sum13/1

== system AvonGasTurbineFAult/thresholds3 ==
  In1 : Inport
  Constant5 : Constant  Value=-0.3406
  Mux5 : Mux  Inputs=3
  Sum12 : Sum  Inputs=|++
  Sum13 : Sum  Inputs=|++
  Sum14 : Sum  Inputs=-+|
  var : Gain  Gain=0.01
  var1 : Gain  Gain=0.19
  Out1 : Outport
  wires:
  In1/1 -> Sum13/1, Mux5/1
  Constant5/1 -> Sum13/2
  Sum12/1 -> Mux5/2
  Mux5/1 -> Out1/1
  var/1 -> Sum12/2, Sum14/1
  Sum13/1 -> Sum14/2, var1/1, Sum12/1
  Sum14/1 -> Mux5/3
  var1/1 -> var/1

== system AvonGasTurbineFAult/thresholds4 ==
  In1 : Inport
  Constant5 : Constant  Value=-2.0766
  Mux5 : Mux  Inputs=3
  Sum12 : Sum  Inputs=|++
  Sum13 : Sum  Inputs=|++
  Sum14 : Sum  Inputs=-+|
  var : Gain  Gain=0.03
  var1 : Gain  Gain=0.19
  Out1 : Outport
  wires:
  var1/1 -> var/1
  Sum14/1 -> Mux5/3
  Sum13/1 -> Sum12/1, var1/1, Sum14/2
  var/1 -> Sum14/1, Sum12/2
  Mux5/1 -> Out1/1
  Sum12/1 -> Mux5/2
  Constant5/1 -> Sum13/2
  In1/1 -> Mux5/1, Sum13/1

== system AvonGasTurbineFAult/thresholds5 ==
  In1 : Inport
  Constant5 : Constant  Value=0
  Mux5 : Mux  Inputs=3
  Sum12 : Sum  Inputs=|++
  Sum13 : Sum  Inputs=|++
  Sum14 : Sum  Inputs=-+|
  var : Gain  Gain=0.25
  var1 : Gain  Gain=0.22
  Out1 : Outport
  wires:
  In1/1 -> Sum13/1, Mux5/1
  Constant5/1 -> Sum13/2
  Sum12/1 -> Mux5/2
  Mux5/1 -> Out1/1
  var/1 -> Sum12/2, Sum14/1
  Sum13/1 -> Sum14/2, var1/1, Sum12/1
  Sum14/1 -> Mux5/3
  var1/1 -> var/1

== system AvonGasTurbineFAult/thresholds6 ==
  In1 : Inport
  Constant5 : Constant  Value=0.0178
  Mux5 : Mux  Inputs=2
  Sum12 : Sum  Inputs=|++
  Sum13 : Sum  Inputs=|++
  Sum14 : Sum  Inputs=-+|
  var : Gain  Gain=0.0665
  var1 : Gain  Gain=0.2
  Out1 : Outport
  wires:
  var1/1 -> var/1
  Sum14/1 -> Mux5/2
  Sum13/1 -> Sum12/1, var1/1, Sum14/2
  var/1 -> Sum14/1, Sum12/2
  Mux5/1 -> Out1/1
  Sum12/1 -> Mux5/1
  Constant5/1 -> Sum13/2
  In1/1 -> Sum13/1

== system AvonGasTurbineFAult/thresholds7 ==
  In1 : Inport
  Constant5 : Constant  Value=-2.9
  Mux5 : Mux  Inputs=2
  Sum12 : Sum  Inputs=|++
  Sum13 : Sum  Inputs=|++
  Sum14 : Sum  Inputs=-+|
  var : Gain  Gain=0.0069
  var1 : Gain  Gain=2.5
  Out1 : Outport
  wires:
  In1/1 -> Sum13/1
  Constant5/1 -> Sum13/2
  Sum12/1 -> Mux5/1
  Mux5/1 -> Out1/1
  var/1 -> Sum12/2, Sum14/1
  Sum13/1 -> Sum14/2, var1/1, Sum12/1
  Sum14/1 -> Mux5/2
  var1/1 -> var/1

== system AvonGasTurbineFAult/thresholds8 ==
  In1 : Inport
  Constant5 : Constant  Value=0.05
  Mux5 : Mux  Inputs=2
  Sum12 : Sum  Inputs=|++
  Sum13 : Sum  Inputs=|++
  Sum14 : Sum  Inputs=-+|
  var : Gain  Gain=0.05
  var1 : Gain  Gain=0.19
  Out1 : Outport
  wires:
  var1/1 -> var/1
  Sum14/1 -> Mux5/2
  Sum13/1 -> Sum12/1, var1/1, Sum14/2
  var/1 -> Sum14/1, Sum12/2
  Mux5/1 -> Out1/1
  Sum12/1 -> Mux5/1
  Constant5/1 -> Sum13/2
  In1/1 -> Sum13/1

== system AvonGasTurbineFAult/thresholds9 ==
  In1 : Inport
  Constant5 : Constant  Value=-0.3406
  Mux5 : Mux  Inputs=2
  Sum12 : Sum  Inputs=|++
  Sum13 : Sum  Inputs=|++
  Sum14 : Sum  Inputs=-+|
  var : Gain  Gain=0.01
  var1 : Gain  Gain=0.19
  Out1 : Outport
  wires:
  In1/1 -> Sum13/1
  Constant5/1 -> Sum13/2
  Sum12/1 -> Mux5/1
  Mux5/1 -> Out1/1
  var/1 -> Sum12/2, Sum14/1
  Sum13/1 -> Sum14/2, var1/1, Sum12/1
  Sum14/1 -> Mux5/2
  var1/1 -> var/1

== system AvonGasTurbineFAult/FG_valve/Layer 1 ==
  "p{1}" : Inport  PortDimensions=6
      mask Display: e = 0.06;c1 = [120 230 180]/255;c2 = ([120 230 180]+0)/(256+128);c3 = ([120 230 180]+128)/(256+128);patch([0 1 1 0],[0 0 1 1],c1);patch([0 1 1 1-e 1-e 0+e],[0 0 1 1-e 0+e 0+e],c2);patch([0 0 1 1-e 0+e 0+e],[0 1 1 1-e 1-e 0+e],c3);plot([0 1 1 0 0],[0 0 1 1 0]);
  Delays 1 : Subsystem
      mask Display: e = 0.06;c1 = [120 150 230]/255;c2 = ([120 150 230]+0)/383;c3 = ([120 150 230]+128)/383;patch([0 1 1 0],[0 0 1 1],c1);patch([0 1 1 1-e 1-e 0+e],[0 0 1 1-e 0+e 0+e],c2);patch([0 0 1 1-e 0+e 0+e],[0 1 1 1-e 1-e 0+e],c3);plot([0 1 1 0 0],[0 0 1 1 0]);disp('0');
  "IW{1,1}" : Subsystem
      mask Display: e = 0.06;c1 = [120 150 230]/255;c2 = ([120 150 230]+0)/383;c3 = ([120 150 230]+128)/383;patch([0 1 1 0],[0 0 1 1],c1);patch([0 1 1 1-e 1-e 0+e],[0 0 1 1-e 0+e 0+e],c2);patch([0 0 1 1-e 0+e 0+e],[0 1 1 1-e 1-e 0+e],c3);plot([0 1 1 0 0],[0 0 1 1 0]);disp('W');
  "b{1}" : Constant  Value=[2.3889224985053104;3.0936934997668795;2.0843855813398791;-3.9744862842578752;-0.0030059466986208966;0.71006181527855206;0.087874090443685549;1.7092387968347751;2.690222447320834;1.5036722448686139]
      mask Display: e = 0.06;c1 = [120 150 230]/255;c2 = ([120 150 230]+0)/383;c3 = ([120 150 230]+128)/383;patch([0 1 1 0],[0 0 1 1],c1);patch([0 1 1 1-e 1-e 0+e],[0 0 1 1-e 0+e 0+e],c2);patch([0 0 1 1-e 0+e 0+e],[0 1 1 1-e 1-e 0+e],c3);plot([0 1 1 0 0],[0 0 1 1 0]);disp('b');
  netsum : Sum  Inputs=2  SaturateOnIntegerOverflow=on  InputSameDT=on  OutDataTypeStr=Inherit: Same as first input
      mask Display: e = 0.06;c1 = [120 150 230]/255;c2 = ([120 150 230]+0)/383;c3 = ([120 150 230]+128)/383;patch([0 1 1 0],[0 0 1 1],c1);patch([0 1 1 1-e 1-e 0+e],[0 0 1 1-e 0+e 0+e],c2);patch([0 0 1 1-e 0+e 0+e],[0 1 1 1-e 1-e 0+e],c3);plot([0 1 1 0 0],[0 0 1 1 0]);disp('+');
  tansig : neural/Transfer Functions/tansig
  "a{1}" : Outport  InitialOutput=[0;0;0;0;0;0;0;0;0;0]
      mask Display: e = 0.06;c1 = [120 230 180]/255;c2 = ([120 230 180]+0)/(256+128);c3 = ([120 230 180]+128)/(256+128);patch([0 1 1 0],[0 0 1 1],c1);patch([0 1 1 1-e 1-e 0+e],[0 0 1 1-e 0+e 0+e],c2);patch([0 0 1 1-e 0+e 0+e],[0 1 1 1-e 1-e 0+e],c3);plot([0 1 1 0 0],[0 0 1 1 0]);
  wires:
  "p{1}"/1 -> Delays 1/1("p{1}")
  Delays 1/1("pd{1,1}") -> "IW{1,1}"/1("pd{1,1}")
  "IW{1,1}"/1("iz{1,1}") -> netsum/1
  "b{1}"/1 -> netsum/2
  netsum/1 -> tansig/1
  tansig/1 -> "a{1}"/1

== system AvonGasTurbineFAult/FG_valve/Layer 2 ==
  "a{1} " : Inport  PortDimensions=10
      mask Display: e = 0.06;c1 = [120 230 180]/255;c2 = ([120 230 180]+0)/(256+128);c3 = ([120 230 180]+128)/(256+128);patch([0 1 1 0],[0 0 1 1],c1);patch([0 1 1 1-e 1-e 0+e],[0 0 1 1-e 0+e 0+e],c2);patch([0 0 1 1-e 0+e 0+e],[0 1 1 1-e 1-e 0+e],c3);plot([0 1 1 0 0],[0 0 1 1 0]);
  Delays 1 : Subsystem
      mask Display: e = 0.06;c1 = [120 150 230]/255;c2 = ([120 150 230]+0)/383;c3 = ([120 150 230]+128)/383;patch([0 1 1 0],[0 0 1 1],c1);patch([0 1 1 1-e 1-e 0+e],[0 0 1 1-e 0+e 0+e],c2);patch([0 0 1 1-e 0+e 0+e],[0 1 1 1-e 1-e 0+e],c3);plot([0 1 1 0 0],[0 0 1 1 0]);disp('0');
  "LW{2,1}" : Subsystem
      mask Display: e = 0.06;c1 = [120 150 230]/255;c2 = ([120 150 230]+0)/383;c3 = ([120 150 230]+128)/383;patch([0 1 1 0],[0 0 1 1],c1);patch([0 1 1 1-e 1-e 0+e],[0 0 1 1-e 0+e 0+e],c2);patch([0 0 1 1-e 0+e 0+e],[0 1 1 1-e 1-e 0+e],c3);plot([0 1 1 0 0],[0 0 1 1 0]);disp('W');
  "b{2}" : Constant  Value=[-1.6910249404990687;-0.25234739619237939;0.29714878476007911;0.73680612754442543;3.145746758476923]
      mask Display: e = 0.06;c1 = [120 150 230]/255;c2 = ([120 150 230]+0)/383;c3 = ([120 150 230]+128)/383;patch([0 1 1 0],[0 0 1 1],c1);patch([0 1 1 1-e 1-e 0+e],[0 0 1 1-e 0+e 0+e],c2);patch([0 0 1 1-e 0+e 0+e],[0 1 1 1-e 1-e 0+e],c3);plot([0 1 1 0 0],[0 0 1 1 0]);disp('b');
  netsum : Sum  Inputs=2  SaturateOnIntegerOverflow=on  InputSameDT=on  OutDataTypeStr=Inherit: Same as first input
      mask Display: e = 0.06;c1 = [120 150 230]/255;c2 = ([120 150 230]+0)/383;c3 = ([120 150 230]+128)/383;patch([0 1 1 0],[0 0 1 1],c1);patch([0 1 1 1-e 1-e 0+e],[0 0 1 1-e 0+e 0+e],c2);patch([0 0 1 1-e 0+e 0+e],[0 1 1 1-e 1-e 0+e],c3);plot([0 1 1 0 0],[0 0 1 1 0]);disp('+');
  softmax : neural/Transfer Functions/softmax
  "a{2}" : Outport  InitialOutput=[0;0;0;0;0]
      mask Display: e = 0.06;c1 = [120 230 180]/255;c2 = ([120 230 180]+0)/(256+128);c3 = ([120 230 180]+128)/(256+128);patch([0 1 1 0],[0 0 1 1],c1);patch([0 1 1 1-e 1-e 0+e],[0 0 1 1-e 0+e 0+e],c2);patch([0 0 1 1-e 0+e 0+e],[0 1 1 1-e 1-e 0+e],c3);plot([0 1 1 0 0],[0 0 1 1 0]);
  wires:
  "a{1} "/1 -> Delays 1/1("p{2}")
  Delays 1/1("pd{2,1}") -> "LW{2,1}"/1("ad{2,1}")
  "LW{2,1}"/1("lz{2,1}") -> netsum/1
  "b{2}"/1 -> netsum/2
  netsum/1 -> softmax/1
  softmax/1 -> "a{2}"/1

== system AvonGasTurbineFAult/FG_valve/Process Input 1 ==
  x : Inport  PortDimensions=6
      mask Display: e = 0.06;c1 = [120 230 180]/255;c2 = ([120 230 180]+0)/(256+128);c3 = ([120 230 180]+128)/(256+128);patch([0 1 1 0],[0 0 1 1],c1);patch([0 1 1 1-e 1-e 0+e],[0 0 1 1-e 0+e 0+e],c2);patch([0 0 1 1-e 0+e 0+e],[0 1 1 1-e 1-e 0+e],c3);plot([0 1 1 0 0],[0 0 1 1 0]);
  mapminmax : neural/Processing Functions/mapminmax  xmin=[-2.6663762834539684;-29.579443895093277;-211.82101487729699;-82.517222745256902;-197.11372544087442;-6.7162251352799531]  xmax=[0.4896409024191879;7.0934102187172812;9.5406620384620737;12.482836129399516;17.146517659039546;2.8792012374116727]  ymin=-1  ymax=1
  p : Outport  PortDimensions=6
      mask Display: e = 0.06;c1 = [120 230 180]/255;c2 = ([120 230 180]+0)/(256+128);c3 = ([120 230 180]+128)/(256+128);patch([0 1 1 0],[0 0 1 1],c1);patch([0 1 1 1-e 1-e 0+e],[0 0 1 1-e 0+e 0+e],c2);patch([0 0 1 1-e 0+e 0+e],[0 1 1 1-e 1-e 0+e],c3);plot([0 1 1 0 0],[0 0 1 1 0]);
  wires:
  x/1 -> mapminmax/1
  mapminmax/1 -> p/1

== system AvonGasTurbineFAult/FG_valve/Process Output 1 ==
  a : Inport  PortDimensions=5
      mask Display: e = 0.06;c1 = [120 230 180]/255;c2 = ([120 230 180]+0)/(256+128);c3 = ([120 230 180]+128)/(256+128);patch([0 1 1 0],[0 0 1 1],c1);patch([0 1 1 1-e 1-e 0+e],[0 0 1 1-e 0+e 0+e],c2);patch([0 0 1 1-e 0+e 0+e],[0 1 1 1-e 1-e 0+e],c3);plot([0 1 1 0 0],[0 0 1 1 0]);
  y : Outport  PortDimensions=5
      mask Display: e = 0.06;c1 = [120 230 180]/255;c2 = ([120 230 180]+0)/(256+128);c3 = ([120 230 180]+128)/(256+128);patch([0 1 1 0],[0 0 1 1],c1);patch([0 1 1 1-e 1-e 0+e],[0 0 1 1-e 0+e 0+e],c2);patch([0 0 1 1-e 0+e 0+e],[0 1 1 1-e 1-e 0+e],c3);plot([0 1 1 0 0],[0 0 1 1 0]);
  wires:
  a/1 -> y/1

== system AvonGasTurbineFAult/IGV/Layer 1 ==
  "p{1}" : Inport  PortDimensions=4
      mask Display: e = 0.06;c1 = [120 230 180]/255;c2 = ([120 230 180]+0)/(256+128);c3 = ([120 230 180]+128)/(256+128);patch([0 1 1 0],[0 0 1 1],c1);patch([0 1 1 1-e 1-e 0+e],[0 0 1 1-e 0+e 0+e],c2);patch([0 0 1 1-e 0+e 0+e],[0 1 1 1-e 1-e 0+e],c3);plot([0 1 1 0 0],[0 0 1 1 0]);
  Delays 1 : Subsystem
      mask Display: e = 0.06;c1 = [120 150 230]/255;c2 = ([120 150 230]+0)/383;c3 = ([120 150 230]+128)/383;patch([0 1 1 0],[0 0 1 1],c1);patch([0 1 1 1-e 1-e 0+e],[0 0 1 1-e 0+e 0+e],c2);patch([0 0 1 1-e 0+e 0+e],[0 1 1 1-e 1-e 0+e],c3);plot([0 1 1 0 0],[0 0 1 1 0]);disp('0');
  "IW{1,1}" : Subsystem
      mask Display: e = 0.06;c1 = [120 150 230]/255;c2 = ([120 150 230]+0)/383;c3 = ([120 150 230]+128)/383;patch([0 1 1 0],[0 0 1 1],c1);patch([0 1 1 1-e 1-e 0+e],[0 0 1 1-e 0+e 0+e],c2);patch([0 0 1 1-e 0+e 0+e],[0 1 1 1-e 1-e 0+e],c3);plot([0 1 1 0 0],[0 0 1 1 0]);disp('W');
  "b{1}" : Constant  Value=[-3.0733170201775559;-3.1113478362828624;2.8379422983871532;5.6668938641369353;-0.32841954150535996;1.9721374550427349;-0.077041183944123293;1.1954965021474624;2.9652126858847145;2.5455900700929619]
      mask Display: e = 0.06;c1 = [120 150 230]/255;c2 = ([120 150 230]+0)/383;c3 = ([120 150 230]+128)/383;patch([0 1 1 0],[0 0 1 1],c1);patch([0 1 1 1-e 1-e 0+e],[0 0 1 1-e 0+e 0+e],c2);patch([0 0 1 1-e 0+e 0+e],[0 1 1 1-e 1-e 0+e],c3);plot([0 1 1 0 0],[0 0 1 1 0]);disp('b');
  netsum : Sum  Inputs=2  SaturateOnIntegerOverflow=on  InputSameDT=on  OutDataTypeStr=Inherit: Same as first input
      mask Display: e = 0.06;c1 = [120 150 230]/255;c2 = ([120 150 230]+0)/383;c3 = ([120 150 230]+128)/383;patch([0 1 1 0],[0 0 1 1],c1);patch([0 1 1 1-e 1-e 0+e],[0 0 1 1-e 0+e 0+e],c2);patch([0 0 1 1-e 0+e 0+e],[0 1 1 1-e 1-e 0+e],c3);plot([0 1 1 0 0],[0 0 1 1 0]);disp('+');
  tansig : neural/Transfer Functions/tansig
  "a{1}" : Outport  InitialOutput=[0;0;0;0;0;0;0;0;0;0]
      mask Display: e = 0.06;c1 = [120 230 180]/255;c2 = ([120 230 180]+0)/(256+128);c3 = ([120 230 180]+128)/(256+128);patch([0 1 1 0],[0 0 1 1],c1);patch([0 1 1 1-e 1-e 0+e],[0 0 1 1-e 0+e 0+e],c2);patch([0 0 1 1-e 0+e 0+e],[0 1 1 1-e 1-e 0+e],c3);plot([0 1 1 0 0],[0 0 1 1 0]);
  wires:
  "p{1}"/1 -> Delays 1/1("p{1}")
  Delays 1/1("pd{1,1}") -> "IW{1,1}"/1("pd{1,1}")
  "IW{1,1}"/1("iz{1,1}") -> netsum/1
  "b{1}"/1 -> netsum/2
  netsum/1 -> tansig/1
  tansig/1 -> "a{1}"/1
